simulink model "emso_teste"  (Simulink 7.1)
settings: Solver=VariableStepDiscrete  StartTime=0.0  StopTime=3.33  RelTol=1e-6
settings Model: Creator=lades  LastModifiedBy=Administrator
settings DataIOCC: ExternalInput=Az
settings DebuggingCC: SolverPrmCheckMsg=none

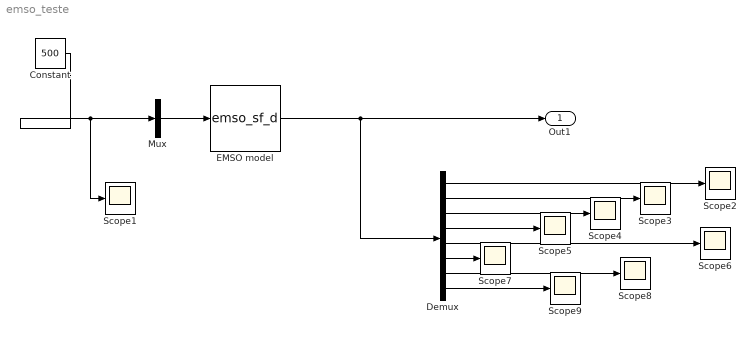
== system emso_teste ==
  Constant : Constant  Value=500  OutDataType=sfix(16)  OutScaling=2^0
  Demux : Demux  Outputs=8
  EMSO model : S-Function  FunctionName=emso_sf_d  Parameters='sample_flash.ems',1,8,0.1  EnableBusSupport=off
  Mux : Mux  Inputs=1
  Scope{1..9} (9 alike) : Scope
      Scope1 settings: TimeRange=2  YMin=4.008258966500001  YMax=4.008258969500001
      Scope2 settings: TimeRange=2  YMin=4.008258966500001  YMax=4.008258969500001
      Scope3 settings: TimeRange=2  YMin=4.008258966500001  YMax=4.008258969500001  SaveName=ScopeData2
      Scope4 settings: TimeRange=2  YMin=4.008258966500001  YMax=4.008258969500001  SaveName=ScopeData3
      Scope5 settings: TimeRange=2  YMin=4.008258966500001  YMax=4.008258969500001  SaveName=ScopeData4
      Scope6 settings: TimeRange=2  YMin=4.008258966500001  YMax=4.008258969500001  SaveName=ScopeData5
      Scope7 settings: TimeRange=2  YMin=4.008258966500001  YMax=4.008258969500001  SaveName=ScopeData6
      Scope8 settings: TimeRange=2  YMin=4.008258966500001  YMax=4.008258969500001  SaveName=ScopeData7
      Scope9 settings: TimeRange=2  YMin=4.008258966500001  YMax=4.008258969500001  SaveName=ScopeData8
  Out1 : Outport  OutDataType=sfix(16)  OutScaling=2^0
  wires:
  EMSO model/1 -> Out1/1, Demux/1
  Mux/1 -> EMSO model/1
  Constant/1 -> Mux/1, Scope1/1
  Demux/1 -> Scope2/1
  Demux/2 -> Scope3/1
  Demux/3 -> Scope4/1
  Demux/4 -> Scope5/1
  Demux/5 -> Scope6/1
  Demux/6 -> Scope7/1
  Demux/7 -> Scope8/1
  Demux/8 -> Scope9/1
